simulink model "Sistema"  (R2023a)
settings: Solver=VariableStepAuto  StartTime=0.0  StopTime=10.0  RelTol=1e-3
settings Model: Creator=isaim  LastModifiedBy=Comgamer
settings DataIOCC: SaveOutput=off  SignalLogging=off  DSMLogging=off  ReturnWorkspaceOutputs=off  TimeSaveName=t
settings DebuggingCC: AlgebraicLoopMsg=none  ArtificialAlgebraicLoopMsg=none  MaxConsecutiveZCsMsg=none  ModelReferenceExtraNoncontSigs=none  OperatingPointInterfaceChecksumMismatchMsg=none

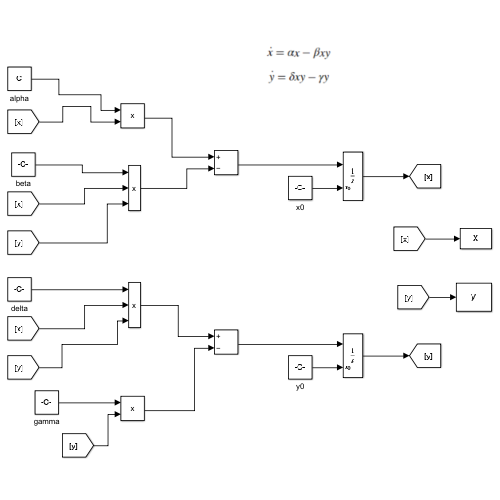
[thumbnail: Simulink's stored preview of the top-level diagram]
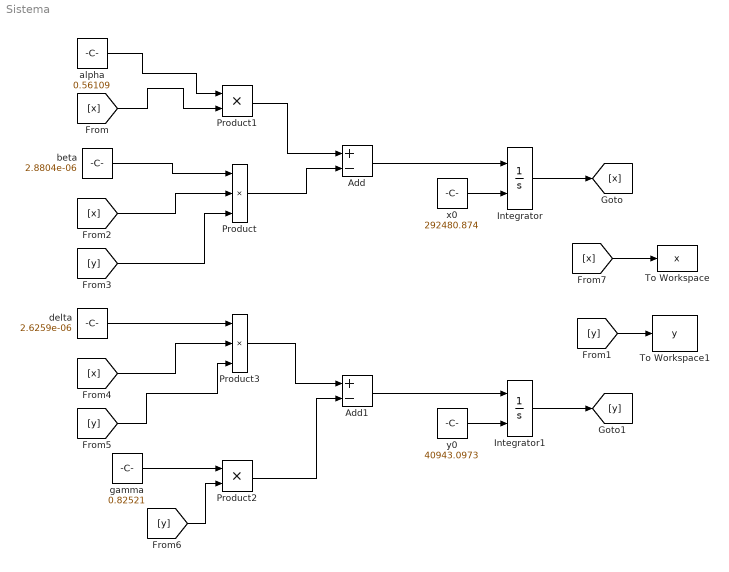
== system Sistema ==
  Add : Sum  Inputs=+-
  Add1 : Sum  Inputs=+-
  Integrator : Integrator  InitialConditionSource=external
  Integrator1 : Integrator  InitialConditionSource=external
  Product : Product  Inputs=3
  Product1 : Product
  Product2 : Product
  Product3 : Product  Inputs=3
  To Workspace : ToWorkspace  VariableName=x  SampleTime=-1
  To Workspace1 : ToWorkspace  VariableName=y  SampleTime=-1
  alpha : Constant  Value=0.56109
  beta : Constant  Value=2.8804e-06
  delta : Constant  Value=2.6259e-06
  gamma : Constant  Value=0.82521
  x0 : Constant  Value=292480.874
  y0 : Constant  Value=40943.0973
  wires:
  Add/1 -> Integrator/1
  Add1/1 -> Integrator1/1
  x0/1 -> Integrator/2
  y0/1 -> Integrator1/2
  Integrator/1 -> [x]
  Integrator1/1 -> [y]
  Product1/1 -> Add/1
  Product/1 -> Add/2
  Product3/1 -> Add1/1
  Product2/1 -> Add1/2
  alpha/1 -> Product1/1
  [x] -> Product1/2
  beta/1 -> Product/1
  [x] -> Product/2
  [y] -> Product/3
  delta/1 -> Product3/1
  [x] -> Product3/2
  [y] -> Product3/3
  gamma/1 -> Product2/1
  [y] -> Product2/2
  [y] -> To Workspace1/1
  [x] -> To Workspace/1
